simulink model "all_afc_0001_0365"  (R2026a)
settings: Solver=ode15s  StopTime=simTime  FixedStep=5e-05  RelTol=1e-06  AbsTol=1e-06
undefined symbols (not defined in the file): AF_sensor_tol, fault_time, fuel_inj_tol, MAF_sensor_tol, measureTime, simTime, spec_num
(part 1 of 3)
Description:
  | Modeling Engine Timing Using Triggered Subsystems
  | 
  | This example presents a model of a four-cylinder spark ignition engine
  | and demonstrates Simulink(R) capabilities to model an internal combustion
  | engine from the throttle to the crankshaft output. We used well-defined
  | physical principles supplemented, where appropriate, with empirical
  | relationships that describe the systems dynamic behavior without
  | introducing unnecessary complexity.
settings Model: ExtModeTrigMode=oneshot  ExtModeArmWhenConnect=off  ExtModeAutoUpdateStatusClock=off  Creator=The MathWorks Inc.  LastModifiedBy=harry_31916
settings SolverCC: ConsecutiveZCsStepRelTol=2.8421709430404e-13
settings DataIOCC: ExternalInput=[t__,u__]  InitialState=[]  LoadExternalInput=on  SaveFormat=StructureWithTime  SignalLoggingSaveFormat=ModelDataLogs  StateSaveName=x  SignalLoggingName=sldemo_engine_output
settings OptimizationCC: BooleanDataType=off  InitFltsAndDblsToZero=on  BufferReusableBoundary=off
settings DebuggingCC: SignalInfNanChecking=warning  SaveWithParameterizedLinksMsg=none  UnderspecifiedInitializationDetection=Classic  SignalResolutionControl=TryResolveAllWithWarning  InheritedTsInSrcMsg=none  MultiTaskDSMMsg=warning  MultiTaskCondExecSysMsg=none  SigSpecEnsureSampleTimeMsg=none  IntegerOverflowMsg=none  ParameterPrecisionLossMsg=none  UniqueDataStoreMsg=warning  IntegerSaturationMsg=none
settings HardwareCC: ProdHWDeviceType=32-bit Generic
settings GRTTargetCC: TargetFcnLib=ansi_tfl_tmw.mat  CombineOutputUpdateFcns=off  GRTInterface=on
settings ConfigComp: CovMetricSettings=d

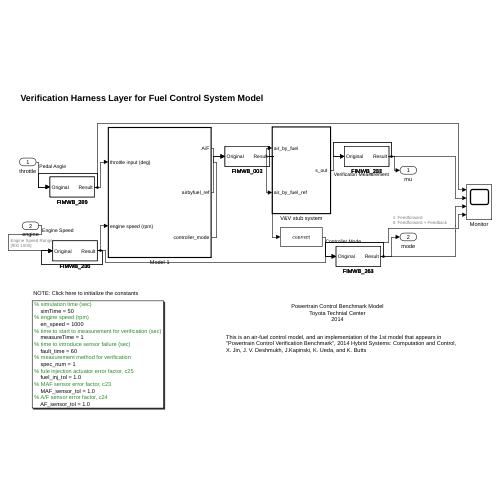
[thumbnail: Simulink's stored preview of the top-level diagram]
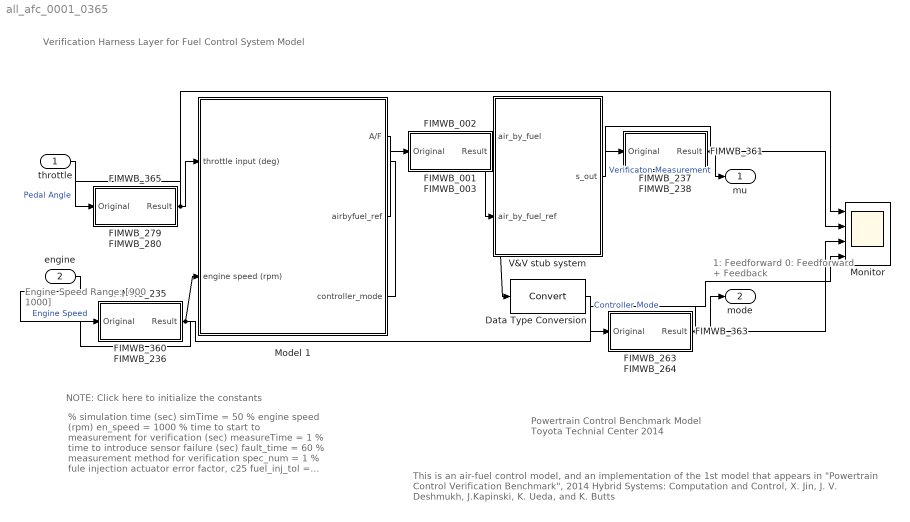
== system all_afc_0001_0365 ==
  note: 1: Feedforward
      | 0: Feedforward + Feedback
  note: NOTE: Click here to initialize the constants
  note: This is an air-fuel control model, and an implementation of the 1st model that appears in
      | "Powertrain Control Verification Benchmark", 2014 Hybrid Systems: Computation and Control,
      | X. Jin, J. V. Deshmukh, J.Kapinski, K. Ueda, and K. Butts
  note: % simulation time (sec)
      |     simTime = 50
      | % engine speed (rpm)
      |     en_speed = 1000
      | % time to start to measurement for verification (sec)
      |     measureTime = 1
      | % time to introduce sensor failure (sec)
      |     fault_time = 60
      | % measurement method for verification
      |     spec_num = 1
      | % fule injection actuator error factor, c25
      |     fuel_inj_tol = 1.0
      | % MAF sensor error factor, c23
      |     MAF_sensor_tol = 1.0
      | % A/F sensor error factor, c24
      |     AF_sensor_tol = 1.0
  note: Engine Speed Range:
      | [900 1000]
  note: Powertrain Control Benchmark Model
      | Toyota Technial Center
      | 2014
  note: Verification Harness Layer for Fuel Control System Model
  throttle : Inport  Interpolate=off
  engine : Inport  Port=2  Interpolate=off
  Data Type Conversion : DataTypeConversion  SaturateOnIntegerOverflow=off  RndMeth=Floor
  FIMWB_001 : Subsystem  Tag=fimwb.fault.1
  FIMWB_002 : Subsystem  Tag=fimwb.fault.2
  FIMWB_003 : Subsystem  Tag=fimwb.fault.3
  FIMWB_235 : Subsystem  Tag=fimwb.fault.235
  FIMWB_236 : Subsystem  Tag=fimwb.fault.236
  FIMWB_237 : Subsystem  Tag=fimwb.fault.237
  FIMWB_238 : Subsystem  Tag=fimwb.fault.238
  FIMWB_263 : Subsystem  Tag=fimwb.fault.263
  FIMWB_264 : Subsystem  Tag=fimwb.fault.264
  FIMWB_279 : Subsystem  Tag=fimwb.fault.279
  FIMWB_280 : Subsystem  Tag=fimwb.fault.280
  FIMWB_360 : Subsystem  Tag=fimwb.fault.360
  FIMWB_361 : Subsystem  Tag=fimwb.fault.361
  FIMWB_363 : Subsystem  Tag=fimwb.fault.363
  FIMWB_365 : Subsystem  Tag=fimwb.fault.365
  Model 1 : Subsystem  Priority=1  TreatAsAtomicUnit=on
  "Monitor " : Scope  NumInputPorts=4
      settings: TimeSpan=50  ActiveDisplayYMinimum=0  ActiveDisplayYMaximum=55
  V&V stub system : Subsystem  TreatAsAtomicUnit=on
  mu : Outport  VectorParamsAs1DForOutWhenUnconnected=off
  mode : Outport  Port=2  VectorParamsAs1DForOutWhenUnconnected=off
  wires:
  engine/1 -> FIMWB_360/1(Original)  "Engine Speed"
  FIMWB_360/1(Result) -> FIMWB_235/1(Original), FIMWB_236/1(Original)
  V&V stub system/1("s_out ") -> FIMWB_361/1(Original)  "Verificaton Measurement"
  FIMWB_361/1(Result) -> FIMWB_237/1(Original), FIMWB_238/1(Original)
  Data Type Conversion/1 -> FIMWB_363/1(Original)  "Controller Mode"
  FIMWB_363/1(Result) -> FIMWB_263/1(Original), FIMWB_264/1(Original)
  throttle/1 -> FIMWB_365/1(Original)  "Pedal Angle"
  FIMWB_365/1(Result) -> FIMWB_279/1(Original), FIMWB_280/1(Original)
  Model 1/1(A/F) -> FIMWB_001/1(Original)
  FIMWB_001/1(Result) -> V&V stub system/1("air_by_fuel ")
  Model 1/2(airbyfuel_ref) -> FIMWB_002/1(Original)
  FIMWB_002/1(Result) -> V&V stub system/2(air_by_fuel_ref)
  Model 1/3(controller_mode) -> FIMWB_003/1(Original)
  FIMWB_003/1(Result) -> Data Type Conversion/1
  FIMWB_235/1(Result) -> "Monitor "/4
  FIMWB_236/1(Result) -> Model 1/2(engine speed (rpm))
  FIMWB_237/1(Result) -> mu/1
  FIMWB_238/1(Result) -> "Monitor "/2
  FIMWB_263/1(Result) -> "Monitor "/3
  FIMWB_264/1(Result) -> mode/1
  FIMWB_279/1(Result) -> "Monitor "/1
  FIMWB_280/1(Result) -> Model 1/1(throttle input (deg))

== system all_afc_0001_0365/FIMWB_001 ==
  Original : Inport
  Result : Outport
  wires:
  Original/1 -> Result/1

== system all_afc_0001_0365/FIMWB_002 ==
  Original : Inport
  Result : Outport
  wires:
  Original/1 -> Result/1

== system all_afc_0001_0365/FIMWB_003 ==
  Original : Inport
  Result : Outport
  wires:
  Original/1 -> Result/1

== system all_afc_0001_0365/FIMWB_235 ==
  Original : Inport
  Result : Outport
  wires:
  Original/1 -> Result/1

== system all_afc_0001_0365/FIMWB_236 ==
  Original : Inport
  Result : Outport
  wires:
  Original/1 -> Result/1

== system all_afc_0001_0365/FIMWB_237 ==
  Original : Inport
  Result : Outport
  wires:
  Original/1 -> Result/1

== system all_afc_0001_0365/FIMWB_238 ==
  Original : Inport
  Result : Outport
  wires:
  Original/1 -> Result/1

== system all_afc_0001_0365/FIMWB_263 ==
  Original : Inport
  Result : Outport
  wires:
  Original/1 -> Result/1

== system all_afc_0001_0365/FIMWB_264 ==
  Original : Inport
  Result : Outport
  wires:
  Original/1 -> Result/1

== system all_afc_0001_0365/FIMWB_279 ==
  Original : Inport
  Result : Outport
  wires:
  Original/1 -> Result/1

== system all_afc_0001_0365/FIMWB_280 ==
  Original : Inport
  Result : Outport
  wires:
  Original/1 -> Result/1

== system all_afc_0001_0365/FIMWB_360 ==
  Original : Inport
  Result : Outport
  wires:
  Original/1 -> Result/1

== system all_afc_0001_0365/FIMWB_361 ==
  Original : Inport
  Result : Outport
  wires:
  Original/1 -> Result/1

== system all_afc_0001_0365/FIMWB_363 ==
  Original : Inport
  Result : Outport
  wires:
  Original/1 -> Result/1

== system all_afc_0001_0365/FIMWB_365 ==
  Original : Inport
  Result : Outport
  wires:
  Original/1 -> Result/1

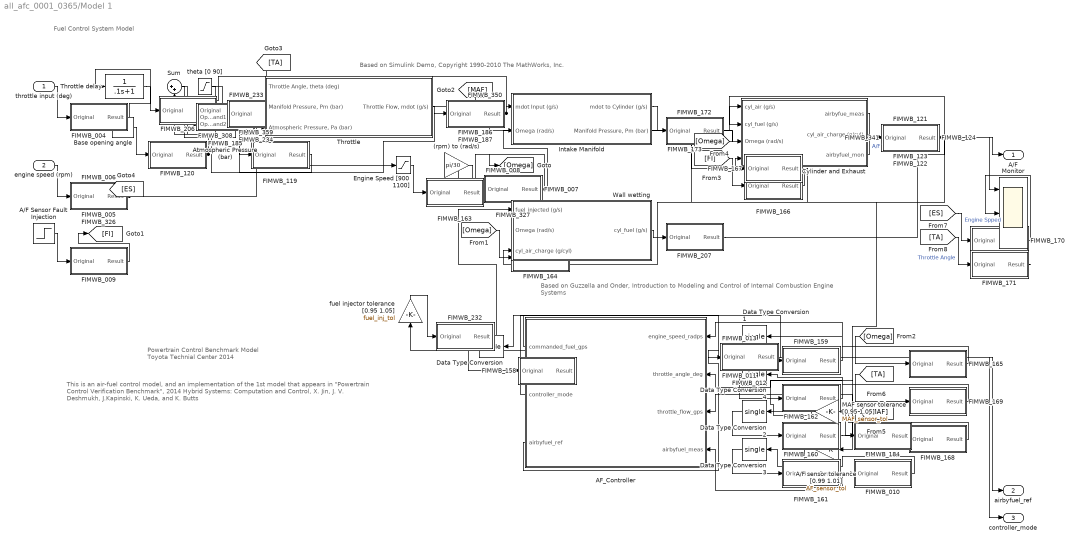
== system all_afc_0001_0365/Model 1 ==
  note: Based on Simulink Demo, Copyright 1990-2010 The MathWorks, Inc.
  note: Based on Guzzella and Onder, Introduction to Modeling and Control of Internal Combustion Engine Systems
  note: Fuel Control System Model
  note: This is an air-fuel control model, and an implementation of the 1st model that appears in
      | "Powertrain Control Verification Benchmark", 2014 Hybrid Systems: Computation and Control,
      | X. Jin, J. V. Deshmukh, J.Kapinski, K. Ueda, and K. Butts
  note: Powertrain Control Benchmark Model
      | Toyota Technial Center
      | 2014
  throttle input (deg) : Inport  Description=[0, 81.2]
      settings: AttributesFormatString=%<Description>
  engine speed (rpm) : Inport  Description=[900,1100]  Port=2
      settings: AttributesFormatString=%<Description>
  (rpm) to (rad/s) : Gain  Gain=pi/30
  A/F Sensor Fault Injection : Step  Time=fault_time  SampleTime=0
      settings: AttributesFormatString=1: Failure\n0: Normal
  A/F sensor tolerance [0.99 1.01] : Gain  Gain=AF_sensor_tol
  AF_Controller : Subsystem  TreatAsAtomicUnit=on
  Atmospheric Pressure (bar) : Constant
  Base opening angle : Constant  Value=8.8
  Cylinder and Exhaust : Subsystem
  Data Type Conversion : DataTypeConversion  OutDataTypeStr=double  SaturateOnIntegerOverflow=off  RndMeth=Floor
  Data Type Conversion{1..4} (4 alike) : DataTypeConversion  OutDataTypeStr=single  SaturateOnIntegerOverflow=off  RndMeth=Floor
  Engine Speed [900 1100] : Saturate  UpperLimit=1100  LowerLimit=900
  FIMWB_004 : Subsystem  Tag=fimwb.fault.4
  FIMWB_005 : Subsystem  Tag=fimwb.fault.5
  FIMWB_006 : Subsystem  Tag=fimwb.fault.6
  FIMWB_007 : Subsystem  Tag=fimwb.fault.7
  FIMWB_008 : Subsystem  Tag=fimwb.fault.8
  FIMWB_009 : Subsystem  Tag=fimwb.fault.9
  FIMWB_010 : Subsystem  Tag=fimwb.fault.10
  FIMWB_011 : Subsystem  Tag=fimwb.fault.11
  FIMWB_012 : Subsystem  Tag=fimwb.fault.12
  FIMWB_013 : Subsystem  Tag=fimwb.fault.13
  FIMWB_119 : Subsystem  Tag=fimwb.fault.119
  FIMWB_120 : Subsystem  Tag=fimwb.fault.120
  FIMWB_121 : Subsystem  Tag=fimwb.fault.121
  FIMWB_122 : Subsystem  Tag=fimwb.fault.122
  FIMWB_123 : Subsystem  Tag=fimwb.fault.123
  FIMWB_124 : Subsystem  Tag=fimwb.fault.124
  FIMWB_158 : Subsystem  Tag=fimwb.fault.158
  FIMWB_159 : Subsystem  Tag=fimwb.fault.159
  FIMWB_160 : Subsystem  Tag=fimwb.fault.160
  FIMWB_161 : Subsystem  Tag=fimwb.fault.161
  FIMWB_162 : Subsystem  Tag=fimwb.fault.162
  FIMWB_163 : Subsystem  Tag=fimwb.fault.163
  FIMWB_164 : Subsystem  Tag=fimwb.fault.164
  FIMWB_165 : Subsystem  Tag=fimwb.fault.165
  FIMWB_166 : Subsystem  Tag=fimwb.fault.166
  FIMWB_167 : Subsystem  Tag=fimwb.fault.167
  FIMWB_168 : Subsystem  Tag=fimwb.fault.168
  FIMWB_169 : Subsystem  Tag=fimwb.fault.169
  FIMWB_170 : Subsystem  Tag=fimwb.fault.170
  FIMWB_171 : Subsystem  Tag=fimwb.fault.171
  FIMWB_172 : Subsystem  Tag=fimwb.fault.172
  FIMWB_173 : Subsystem  Tag=fimwb.fault.173
  FIMWB_184 : Subsystem  Tag=fimwb.fault.184
  FIMWB_185 : Subsystem  Tag=fimwb.fault.185
  FIMWB_186 : Subsystem  Tag=fimwb.fault.186
  FIMWB_187 : Subsystem  Tag=fimwb.fault.187
  FIMWB_206 : Subsystem  Tag=fimwb.fault.206
  FIMWB_207 : Subsystem  Tag=fimwb.fault.207
  FIMWB_232 : Subsystem  Tag=fimwb.fault.232
  FIMWB_233 : Subsystem  Tag=fimwb.fault.233
  FIMWB_234 : Subsystem  Tag=fimwb.fault.234
  FIMWB_308 : Subsystem  Tag=fimwb.fault.308
  FIMWB_326 : Subsystem  Tag=fimwb.fault.326
  FIMWB_327 : Subsystem  Tag=fimwb.fault.327
  FIMWB_341 : Subsystem  Tag=fimwb.fault.341
  FIMWB_350 : Subsystem  Tag=fimwb.fault.350
  FIMWB_359 : Subsystem  Tag=fimwb.fault.359
  Intake Manifold : Subsystem
  MAF sensor tolerance [0.95 1.05] : Gain  Gain=MAF_sensor_tol
  Monitor : Scope  NumInputPorts=3
      settings: TimeSpan=85  ActiveDisplayYMinimum=11.75  ActiveDisplayYMaximum=14.75
  Sum : Sum  Inputs=|++
  Throttle : Subsystem
  Throttle delay : TransferFcn  Denominator=[.1 1]
  Wall wetting : Subsystem
  fuel injector tolerance [0.95 1.05] : Gain  Gain=fuel_inj_tol
  theta [0 90] : Saturate  UpperLimit=90  LowerLimit=0
  A/F : Outport  VectorParamsAs1DForOutWhenUnconnected=off
  airbyfuel_ref : Outport  Port=2  VectorParamsAs1DForOutWhenUnconnected=off
  controller_mode : Outport  Port=3  VectorParamsAs1DForOutWhenUnconnected=off
  wires:
  Sum/1 -> FIMWB_308/1(Original)
  engine speed (rpm)/1 -> FIMWB_326/1(Original)
  FIMWB_326/1(Result) -> FIMWB_005/1(Original), FIMWB_006/1(Original)
  (rpm) to (rad/s)/1 -> FIMWB_327/1(Original)
  FIMWB_327/1(Result) -> FIMWB_007/1(Original), FIMWB_008/1(Original)
  Cylinder and Exhaust/3("airbyfuel_mon ") -> FIMWB_341/1(Original)  "A/F"
  FIMWB_341/1(Result) -> FIMWB_123/1(Original), FIMWB_124/1(Original)
  Throttle/1("Throttle Flow, mdot (g/s)") -> FIMWB_350/1(Original)
  FIMWB_350/1(Result) -> FIMWB_186/1(Original), FIMWB_187/1(Original)
  theta [0 90]/1 -> FIMWB_359/1(Original)
  FIMWB_359/1(Result) -> FIMWB_233/1(Original), FIMWB_234/1(Original)
  throttle input (deg)/1 -> FIMWB_004/1(Original)
  FIMWB_004/1(Result) -> Throttle delay/1
  FIMWB_005/1(Result) -> Engine Speed [900 1100]/1
  FIMWB_006/1(Result) -> [ES]
  FIMWB_007/1(Result) -> [Omega]
  FIMWB_008/1(Result) -> Intake Manifold/2(Omega (rad/s))
  A/F Sensor Fault Injection/1 -> FIMWB_009/1(Original)
  FIMWB_009/1(Result) -> [FI]
  A/F sensor tolerance [0.99 1.01]/1 -> FIMWB_010/1(Original)
  FIMWB_010/1(Result) -> Data Type Conversion3/1
  AF_Controller/1(commanded_fuel_gps) -> FIMWB_011/1(Original)
  FIMWB_011/1(Result) -> Data Type Conversion/1
  AF_Controller/2(controller_mode) -> FIMWB_012/1(Original)
  FIMWB_012/1(Result) -> controller_mode/1
  AF_Controller/3(airbyfuel_ref) -> FIMWB_013/1(Original)
  FIMWB_013/1(Result) -> airbyfuel_ref/1
  Atmospheric Pressure (bar)/1 -> FIMWB_119/1(Original)
  FIMWB_119/1(Result) -> Throttle/3("Atmospheric Pressure, Pa (bar) ")
  Base opening angle/1 -> FIMWB_120/1(Original)
  FIMWB_120/1(Result) -> Sum/2, FIMWB_308/3(Operand2)
  Cylinder and Exhaust/1(airbyfue_meas) -> FIMWB_121/1(Original)
  FIMWB_121/1(Result) -> A/F sensor tolerance [0.99 1.01]/1
  Cylinder and Exhaust/2(cyl_air_charge (g/cyl)) -> FIMWB_122/1(Original)
  FIMWB_122/1(Result) -> Wall wetting/3(cyl_air_charge (g/cyl))
  FIMWB_123/1(Result) -> Monitor/1
  FIMWB_124/1(Result) -> A/F/1
  Data Type Conversion/1 -> FIMWB_158/1(Original)
  FIMWB_158/1(Result) -> fuel injector tolerance [0.95 1.05]/1
  Data Type Conversion1/1 -> FIMWB_159/1(Original)
  FIMWB_159/1(Result) -> AF_Controller/1(engine_speed_radps)
  Data Type Conversion2/1 -> FIMWB_160/1(Original)
  FIMWB_160/1(Result) -> AF_Controller/3(throttle_flow_gps)
  Data Type Conversion3/1 -> FIMWB_161/1(Original)
  FIMWB_161/1(Result) -> AF_Controller/4(airbyfuel_meas)
  Data Type Conversion4/1 -> FIMWB_162/1(Original)
  FIMWB_162/1(Result) -> AF_Controller/2(throttle_angle_deg)
  Engine Speed [900 1100]/1 -> FIMWB_163/1(Original)
  FIMWB_163/1(Result) -> (rpm) to (rad/s)/1
  [Omega] -> FIMWB_164/1(Original)
  FIMWB_164/1(Result) -> Wall wetting/2(Omega (rad/s))
  [Omega] -> FIMWB_165/1(Original)
  FIMWB_165/1(Result) -> Data Type Conversion1/1
  [FI] -> FIMWB_166/1(Original)
  FIMWB_166/1(Result) -> Cylinder and Exhaust/4(SensorFault)
  [Omega] -> FIMWB_167/1(Original)
  FIMWB_167/1(Result) -> Cylinder and Exhaust/3(Omega (rad/s))
  [MAF] -> FIMWB_168/1(Original)
  FIMWB_168/1(Result) -> MAF sensor tolerance [0.95 1.05]/1
  [TA] -> FIMWB_169/1(Original)
  FIMWB_169/1(Result) -> Data Type Conversion4/1
  [ES] -> FIMWB_170/1(Original)  "Engine Spped"
  FIMWB_170/1(Result) -> Monitor/2
  [TA] -> FIMWB_171/1(Original)  "Throttle Angle"
  FIMWB_171/1(Result) -> Monitor/3
  Intake Manifold/1(mdot to Cylinder (g/s)) -> FIMWB_172/1(Original)
  FIMWB_172/1(Result) -> Cylinder and Exhaust/1(cyl_air (g/s))
  Intake Manifold/2("Manifold Pressure, Pm (bar)") -> FIMWB_173/1(Original)
  FIMWB_173/1(Result) -> Throttle/2("Manifold Pressure, Pm (bar)")
  MAF sensor tolerance [0.95 1.05]/1 -> FIMWB_184/1(Original)
  FIMWB_184/1(Result) -> Data Type Conversion2/1
  FIMWB_308/1(Result) -> FIMWB_185/1(Original)
  FIMWB_185/1(Result) -> theta [0 90]/1
  FIMWB_186/1(Result) -> [MAF]
  FIMWB_187/1(Result) -> Intake Manifold/1(mdot Input (g/s))
  Throttle delay/1 -> FIMWB_206/1(Original)
  FIMWB_206/1(Result) -> Sum/1, FIMWB_308/2(Operand1)
  Wall wetting/1(cyl_fuel (g/s)) -> FIMWB_207/1(Original)
  FIMWB_207/1(Result) -> Cylinder and Exhaust/2(cyl_fuel (g/s))
  fuel injector tolerance [0.95 1.05]/1 -> FIMWB_232/1(Original)
  FIMWB_232/1(Result) -> Wall wetting/1(fuel_injected (g/s))
  FIMWB_233/1(Result) -> [TA]
  FIMWB_234/1(Result) -> Throttle/1("Throttle Angle, theta (deg)")

== system all_afc_0001_0365/V&V stub system ==
  "air_by_fuel " : Inport  OutDataTypeStr=double
  air_by_fuel_ref : Inport  Port=2
  Calcuate Error : Subsystem  Priority=20  TreatAsAtomicUnit=on
  Constant : Constant  Value=0.5
  Data Type Conversion : DataTypeConversion  OutDataTypeStr=double  SaturateOnIntegerOverflow=off  RndMeth=Floor
  FIMWB_239 : Subsystem  Tag=fimwb.fault.239
  FIMWB_240 : Subsystem  Tag=fimwb.fault.240
  FIMWB_260 : Subsystem  Tag=fimwb.fault.260
  FIMWB_261 : Subsystem  Tag=fimwb.fault.261
  FIMWB_265 : Subsystem  Tag=fimwb.fault.265
  FIMWB_275 : Subsystem  Tag=fimwb.fault.275
  FIMWB_276 : Subsystem  Tag=fimwb.fault.276
  MeasureOn : Step  Time=measureTime  SampleTime=0
  Relational Operator : RelationalOperator  Operator=>  OutDataTypeStr=boolean  InputSameDT=off
  spec_num : Constant  Value=spec_num  OutDataTypeStr=uint8
  "s_out " : Outport  VectorParamsAs1DForOutWhenUnconnected=off
  wires:
  Relational Operator/1 -> Calcuate Error/Enable
  "air_by_fuel "/1 -> FIMWB_239/1(Original)
  FIMWB_239/1(Result) -> Calcuate Error/1("air_by_fuel ")
  Calcuate Error/1("s_out ") -> FIMWB_240/1(Original)
  FIMWB_240/1(Result) -> "s_out "/1
  Constant/1 -> FIMWB_260/1(Original)
  FIMWB_260/1(Result) -> Relational Operator/2
  MeasureOn/1 -> FIMWB_261/1(Original)
  FIMWB_261/1(Result) -> Relational Operator/1
  spec_num/1 -> FIMWB_265/1(Original)
  FIMWB_265/1(Result) -> Calcuate Error/2(spec_num)
  air_by_fuel_ref/1 -> FIMWB_275/1(Original)
  FIMWB_275/1(Result) -> Data Type Conversion/1
  Data Type Conversion/1 -> FIMWB_276/1(Original)
  FIMWB_276/1(Result) -> Calcuate Error/3(air_by_fuel_ref)

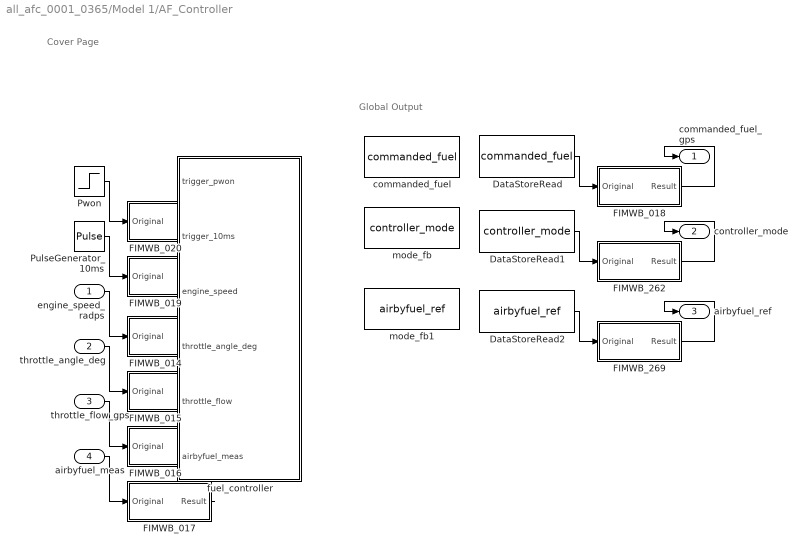
== system all_afc_0001_0365/Model 1/AF_Controller ==
  note: Global Output
  note: Cover Page
  engine_speed_radps : Inport
  throttle_angle_deg : Inport  Port=2
  throttle_flow_gps : Inport  Port=3
  airbyfuel_meas : Inport  Port=4
  DataStoreRead : DataStoreRead  Priority=2  DataStoreName=commanded_fuel  IndexOptions=Index vector (dialog)  Indices=1  OutputSizes=1
  DataStoreRead1 : DataStoreRead  Priority=2  DataStoreName=controller_mode  IndexOptions=Index vector (dialog)  Indices=1  OutputSizes=1
  DataStoreRead2 : DataStoreRead  Priority=2  DataStoreName=airbyfuel_ref  IndexOptions=Index vector (dialog)  Indices=1  OutputSizes=1
  FIMWB_014 : Subsystem  Tag=fimwb.fault.14
  FIMWB_015 : Subsystem  Tag=fimwb.fault.15
  FIMWB_016 : Subsystem  Tag=fimwb.fault.16
  FIMWB_017 : Subsystem  Tag=fimwb.fault.17
  FIMWB_018 : Subsystem  Tag=fimwb.fault.18
  FIMWB_019 : Subsystem  Tag=fimwb.fault.19
  FIMWB_020 : Subsystem  Tag=fimwb.fault.20
  FIMWB_262 : Subsystem  Tag=fimwb.fault.262
  FIMWB_269 : Subsystem  Tag=fimwb.fault.269
  PulseGenerator_10ms : DiscretePulseGenerator  PulseType=Time based  Period=0.01  PulseWidth=50  PhaseDelay=0.01
  Pwon : Step  Time=0.001  SampleTime=0
  commanded_fuel : DataStoreMemory  DataStoreName=commanded_fuel  InitialValue=0.1726  ShowAdditionalParam=off  OutDataTypeStr=single
      settings: AttributesFormatString=commanded_fuel
  fuel_controller : Subsystem  Priority=1  TreatAsAtomicUnit=on
      settings: AttributesFormatString=Priority = %<Priority>
  mode_fb : DataStoreMemory  DataStoreName=controller_mode  ShowAdditionalParam=off  OutDataTypeStr=boolean
      settings: AttributesFormatString=controller_mode
  mode_fb1 : DataStoreMemory  DataStoreName=airbyfuel_ref  ShowAdditionalParam=off  OutDataTypeStr=single
  commanded_fuel_gps : Outport  VectorParamsAs1DForOutWhenUnconnected=off
  controller_mode : Outport  Port=2  VectorParamsAs1DForOutWhenUnconnected=off
  airbyfuel_ref : Outport  Port=3  VectorParamsAs1DForOutWhenUnconnected=off
  wires:
  engine_speed_radps/1 -> FIMWB_014/1(Original)
  FIMWB_014/1(Result) -> fuel_controller/3(engine_speed)
  throttle_angle_deg/1 -> FIMWB_015/1(Original)
  FIMWB_015/1(Result) -> fuel_controller/4(throttle_angle_deg)
  throttle_flow_gps/1 -> FIMWB_016/1(Original)
  FIMWB_016/1(Result) -> fuel_controller/5(throttle_flow)
  airbyfuel_meas/1 -> FIMWB_017/1(Original)
  FIMWB_017/1(Result) -> fuel_controller/6(airbyfuel_meas)
  DataStoreRead/1 -> FIMWB_018/1(Original)
  FIMWB_018/1(Result) -> commanded_fuel_gps/1
  PulseGenerator_10ms/1 -> FIMWB_019/1(Original)
  FIMWB_019/1(Result) -> fuel_controller/2(trigger_10ms)
  Pwon/1 -> FIMWB_020/1(Original)
  FIMWB_020/1(Result) -> fuel_controller/1(trigger_pwon)
  DataStoreRead1/1 -> FIMWB_262/1(Original)
  FIMWB_262/1(Result) -> controller_mode/1
  DataStoreRead2/1 -> FIMWB_269/1(Original)
  FIMWB_269/1(Result) -> airbyfuel_ref/1

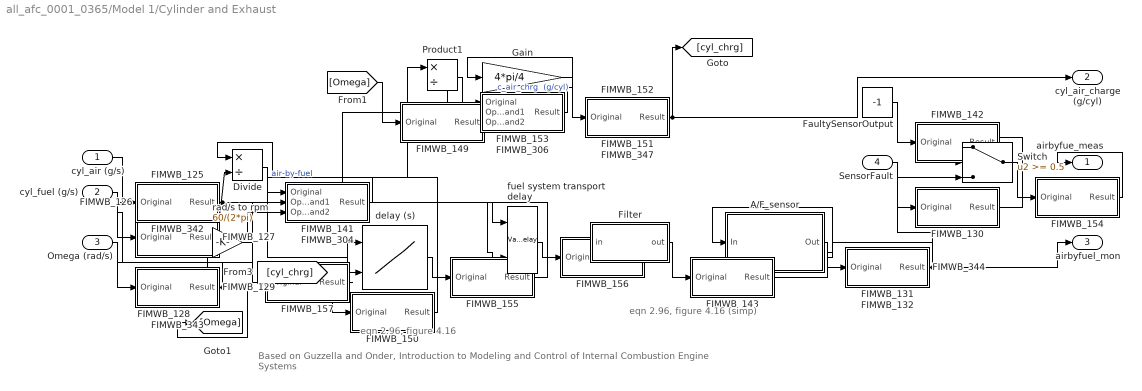
== system all_afc_0001_0365/Model 1/Cylinder and Exhaust ==
  note: Based on Guzzella and Onder, Introduction to Modeling and Control of Internal Combustion Engine Systems
  note: eqn 2.96, figure 4.16
  note: eqn 2.96, figure 4.16 (simp)
  cyl_air (g/s) : Inport
  cyl_fuel (g/s) : Inport  Port=2
  Omega (rad/s) : Inport  Port=3
  SensorFault : Inport  Port=4
  A/F_sensor : Subsystem
  Divide : Product  Inputs=*/
  FIMWB_125 : Subsystem  Tag=fimwb.fault.125
  FIMWB_126 : Subsystem  Tag=fimwb.fault.126
  FIMWB_127 : Subsystem  Tag=fimwb.fault.127
  FIMWB_128 : Subsystem  Tag=fimwb.fault.128
  FIMWB_129 : Subsystem  Tag=fimwb.fault.129
  FIMWB_130 : Subsystem  Tag=fimwb.fault.130
  FIMWB_131 : Subsystem  Tag=fimwb.fault.131
  FIMWB_132 : Subsystem  Tag=fimwb.fault.132
  FIMWB_141 : Subsystem  Tag=fimwb.fault.141
  FIMWB_142 : Subsystem  Tag=fimwb.fault.142
  FIMWB_143 : Subsystem  Tag=fimwb.fault.143
  FIMWB_149 : Subsystem  Tag=fimwb.fault.149
  FIMWB_150 : Subsystem  Tag=fimwb.fault.150
  FIMWB_151 : Subsystem  Tag=fimwb.fault.151
  FIMWB_152 : Subsystem  Tag=fimwb.fault.152
  FIMWB_153 : Subsystem  Tag=fimwb.fault.153
  FIMWB_154 : Subsystem  Tag=fimwb.fault.154
  FIMWB_155 : Subsystem  Tag=fimwb.fault.155
  FIMWB_156 : Subsystem  Tag=fimwb.fault.156
  FIMWB_157 : Subsystem  Tag=fimwb.fault.157
  FIMWB_304 : Subsystem  Tag=fimwb.fault.304
  FIMWB_306 : Subsystem  Tag=fimwb.fault.306
  FIMWB_342 : Subsystem  Tag=fimwb.fault.342
  FIMWB_343 : Subsystem  Tag=fimwb.fault.343
  FIMWB_344 : Subsystem  Tag=fimwb.fault.344
  FIMWB_347 : Subsystem  Tag=fimwb.fault.347
  FaultySensorOutput : Constant  Value=-1
  Filter : Subsystem
  Gain : Gain  Gain=4*pi/4
  Product1 : Product  Inputs=*/  RndMeth=Zero
  Switch : Switch  Threshold=0.5  SaturateOnIntegerOverflow=off  InputSameDT=off
  delay (s) : Lookup_n-D  BreakpointsForDimension1=[800,1000,1500,2000,3000]  BreakpointsForDimension2=[0.05,0.15,0.2,0.25]  Table=reshape([0.8,0.6,0.4,0.3,0.2,0.4,0.3,0.2,0.2,0.2,0.3,0.25,0.2,0.2,0.2,0.25,0.2,0.2,0.2,0.2],5,4)  UseLastTableValue=on  RndMeth=Simplest
      settings: InputPortMap=u0,u1
  fuel system transport delay : VariableTransportDelay  VariableDelayType=Variable transport delay  MaximumDelay=10  InitialOutput=14.7  MaximumPoints=20480
  rad/s to rpm : Gain  Gain=60/(2*pi)
  airbyfue_meas : Outport  VectorParamsAs1DForOutWhenUnconnected=off
  cyl_air_charge (g/cyl) : Outport  Port=2  VectorParamsAs1DForOutWhenUnconnected=off
  "airbyfuel_mon " : Outport  Port=3  VectorParamsAs1DForOutWhenUnconnected=off
  wires:
  Divide/1 -> FIMWB_304/1(Original)  "air-by-fuel"
  Product1/1 -> FIMWB_306/1(Original)
  cyl_air (g/s)/1 -> FIMWB_342/1(Original)
  FIMWB_342/1(Result) -> FIMWB_125/1(Original), FIMWB_126/1(Original)
  Omega (rad/s)/1 -> FIMWB_343/1(Original)
  FIMWB_343/1(Result) -> FIMWB_128/1(Original), FIMWB_129/1(Original)
  A/F_sensor/1(Out) -> FIMWB_344/1(Original)
  FIMWB_344/1(Result) -> FIMWB_131/1(Original), FIMWB_132/1(Original)
  Gain/1 -> FIMWB_347/1(Original)  "c_air_chrg  (g/cyl)"
  FIMWB_347/1(Result) -> FIMWB_151/1(Original), FIMWB_152/1(Original)
  FIMWB_125/1(Result) -> Divide/1, FIMWB_304/2(Operand1)
  FIMWB_126/1(Result) -> Product1/1, FIMWB_306/2(Operand1)
  cyl_fuel (g/s)/1 -> FIMWB_127/1(Original)
  FIMWB_127/1(Result) -> Divide/2, FIMWB_304/3(Operand2)
  FIMWB_128/1(Result) -> [Omega]
  FIMWB_129/1(Result) -> rad/s to rpm/1
  SensorFault/1 -> FIMWB_130/1(Original)
  FIMWB_130/1(Result) -> Switch/2
  FIMWB_131/1(Result) -> Switch/3
  FIMWB_132/1(Result) -> "airbyfuel_mon "/1
  FIMWB_304/1(Result) -> FIMWB_141/1(Original)
  FIMWB_141/1(Result) -> fuel system transport delay/1
  FaultySensorOutput/1 -> FIMWB_142/1(Original)
  FIMWB_142/1(Result) -> Switch/1
  Filter/1(out) -> FIMWB_143/1(Original)
  FIMWB_143/1(Result) -> A/F_sensor/1(In)
  [Omega] -> FIMWB_149/1(Original)
  FIMWB_149/1(Result) -> Product1/2, FIMWB_306/3(Operand2)
  [cyl_chrg] -> FIMWB_150/1(Original)
  FIMWB_150/1(Result) -> delay (s)/2
  FIMWB_151/1(Result) -> [cyl_chrg]
  FIMWB_152/1(Result) -> cyl_air_charge (g/cyl)/1
  FIMWB_306/1(Result) -> FIMWB_153/1(Original)
  FIMWB_153/1(Result) -> Gain/1
  Switch/1 -> FIMWB_154/1(Original)
  FIMWB_154/1(Result) -> airbyfue_meas/1
  delay (s)/1 -> FIMWB_155/1(Original)
  FIMWB_155/1(Result) -> fuel system transport delay/2
  fuel system transport delay/1 -> FIMWB_156/1(Original)
  FIMWB_156/1(Result) -> Filter/1(in)
  rad/s to rpm/1 -> FIMWB_157/1(Original)
  FIMWB_157/1(Result) -> delay (s)/1

== system all_afc_0001_0365/Model 1/FIMWB_004 ==
  Original : Inport
  Result : Outport
  wires:
  Original/1 -> Result/1

== system all_afc_0001_0365/Model 1/FIMWB_005 ==
  Original : Inport
  Result : Outport
  wires:
  Original/1 -> Result/1

== system all_afc_0001_0365/Model 1/FIMWB_006 ==
  Original : Inport
  Result : Outport
  wires:
  Original/1 -> Result/1

== system all_afc_0001_0365/Model 1/FIMWB_007 ==
  Original : Inport
  Result : Outport
  wires:
  Original/1 -> Result/1

== system all_afc_0001_0365/Model 1/FIMWB_008 ==
  Original : Inport
  Result : Outport
  wires:
  Original/1 -> Result/1

== system all_afc_0001_0365/Model 1/FIMWB_009 ==
  Original : Inport
  Result : Outport
  wires:
  Original/1 -> Result/1

== system all_afc_0001_0365/Model 1/FIMWB_010 ==
  Original : Inport
  Result : Outport
  wires:
  Original/1 -> Result/1

== system all_afc_0001_0365/Model 1/FIMWB_011 ==
  Original : Inport
  Result : Outport
  wires:
  Original/1 -> Result/1

== system all_afc_0001_0365/Model 1/FIMWB_012 ==
  Original : Inport
  Result : Outport
  wires:
  Original/1 -> Result/1

== system all_afc_0001_0365/Model 1/FIMWB_013 ==
  Original : Inport
  Result : Outport
  wires:
  Original/1 -> Result/1

== system all_afc_0001_0365/Model 1/FIMWB_119 ==
  Original : Inport
  Result : Outport
  wires:
  Original/1 -> Result/1

== system all_afc_0001_0365/Model 1/FIMWB_120 ==
  Original : Inport
  Result : Outport
  wires:
  Original/1 -> Result/1

== system all_afc_0001_0365/Model 1/FIMWB_121 ==
  Original : Inport
  Result : Outport
  wires:
  Original/1 -> Result/1

== system all_afc_0001_0365/Model 1/FIMWB_122 ==
  Original : Inport
  Result : Outport
  wires:
  Original/1 -> Result/1

== system all_afc_0001_0365/Model 1/FIMWB_123 ==
  Original : Inport
  Result : Outport
  wires:
  Original/1 -> Result/1

== system all_afc_0001_0365/Model 1/FIMWB_124 ==
  Original : Inport
  Result : Outport
  wires:
  Original/1 -> Result/1

== system all_afc_0001_0365/Model 1/FIMWB_158 ==
  Original : Inport
  Result : Outport
  wires:
  Original/1 -> Result/1

== system all_afc_0001_0365/Model 1/FIMWB_159 ==
  Original : Inport
  Result : Outport
  wires:
  Original/1 -> Result/1

== system all_afc_0001_0365/Model 1/FIMWB_160 ==
  Original : Inport
  Result : Outport
  wires:
  Original/1 -> Result/1

== system all_afc_0001_0365/Model 1/FIMWB_161 ==
  Original : Inport
  Result : Outport
  wires:
  Original/1 -> Result/1

== system all_afc_0001_0365/Model 1/FIMWB_162 ==
  Original : Inport
  Result : Outport
  wires:
  Original/1 -> Result/1

== system all_afc_0001_0365/Model 1/FIMWB_163 ==
  Original : Inport
  Result : Outport
  wires:
  Original/1 -> Result/1

== system all_afc_0001_0365/Model 1/FIMWB_164 ==
  Original : Inport
  Result : Outport
  wires:
  Original/1 -> Result/1

== system all_afc_0001_0365/Model 1/FIMWB_165 ==
  Original : Inport
  Result : Outport
  wires:
  Original/1 -> Result/1

== system all_afc_0001_0365/Model 1/FIMWB_166 ==
  Original : Inport
  Result : Outport
  wires:
  Original/1 -> Result/1

== system all_afc_0001_0365/Model 1/FIMWB_167 ==
  Original : Inport
  Result : Outport
  wires:
  Original/1 -> Result/1

== system all_afc_0001_0365/Model 1/FIMWB_168 ==
  Original : Inport
  Result : Outport
  wires:
  Original/1 -> Result/1

== system all_afc_0001_0365/Model 1/FIMWB_169 ==
  Original : Inport
  Result : Outport
  wires:
  Original/1 -> Result/1

== system all_afc_0001_0365/Model 1/FIMWB_170 ==
  Original : Inport
  Result : Outport
  wires:
  Original/1 -> Result/1

== system all_afc_0001_0365/Model 1/FIMWB_171 ==
  Original : Inport
  Result : Outport
  wires:
  Original/1 -> Result/1

== system all_afc_0001_0365/Model 1/FIMWB_172 ==
  Original : Inport
  Result : Outport
  wires:
  Original/1 -> Result/1

== system all_afc_0001_0365/Model 1/FIMWB_173 ==
  Original : Inport
  Result : Outport
  wires:
  Original/1 -> Result/1

== system all_afc_0001_0365/Model 1/FIMWB_184 ==
  Original : Inport
  Result : Outport
  wires:
  Original/1 -> Result/1

== system all_afc_0001_0365/Model 1/FIMWB_185 ==
  Original : Inport
  Result : Outport
  wires:
  Original/1 -> Result/1

== system all_afc_0001_0365/Model 1/FIMWB_186 ==
  Original : Inport
  Result : Outport
  wires:
  Original/1 -> Result/1

== system all_afc_0001_0365/Model 1/FIMWB_187 ==
  Original : Inport
  Result : Outport
  wires:
  Original/1 -> Result/1

== system all_afc_0001_0365/Model 1/FIMWB_206 ==
  Original : Inport
  Result : Outport
  wires:
  Original/1 -> Result/1

== system all_afc_0001_0365/Model 1/FIMWB_207 ==
  Original : Inport
  Result : Outport
  wires:
  Original/1 -> Result/1

== system all_afc_0001_0365/Model 1/FIMWB_232 ==
  Original : Inport
  Result : Outport
  wires:
  Original/1 -> Result/1

== system all_afc_0001_0365/Model 1/FIMWB_233 ==
  Original : Inport
  Result : Outport
  wires:
  Original/1 -> Result/1

== system all_afc_0001_0365/Model 1/FIMWB_234 ==
  Original : Inport
  Result : Outport
  wires:
  Original/1 -> Result/1

== system all_afc_0001_0365/Model 1/FIMWB_308 ==
  Original : Inport
  Operand1 : Inport  Port=2
  Operand2 : Inport  Port=3
  Unused2 : Terminator
  Unused3 : Terminator
  Result : Outport
  wires:
  Original/1 -> Result/1
  Operand1/1 -> Unused2/1
  Operand2/1 -> Unused3/1

== system all_afc_0001_0365/Model 1/FIMWB_326 ==
  Original : Inport
  Result : Outport
  wires:
  Original/1 -> Result/1

== system all_afc_0001_0365/Model 1/FIMWB_327 ==
  Original : Inport
  Result : Outport
  wires:
  Original/1 -> Result/1

== system all_afc_0001_0365/Model 1/FIMWB_341 ==
  Original : Inport
  Result : Outport
  wires:
  Original/1 -> Result/1

== system all_afc_0001_0365/Model 1/FIMWB_350 ==
  Original : Inport
  Result : Outport
  wires:
  Original/1 -> Result/1

== system all_afc_0001_0365/Model 1/FIMWB_359 ==
  Original : Inport
  Result : Outport
  wires:
  Original/1 -> Result/1

== system all_afc_0001_0365/Model 1/Intake Manifold ==
  note: Intake Manifold Vacuum
  note: Based on Simulink Demo, Copyright 1990-2010 The MathWorks, Inc.
  mdot Input (g/s) : Inport
  Omega (rad/s) : Inport  Port=2
  FIMWB_174 : Subsystem  Tag=fimwb.fault.174
  FIMWB_175 : Subsystem  Tag=fimwb.fault.175
  FIMWB_176 : Subsystem  Tag=fimwb.fault.176
  FIMWB_177 : Subsystem  Tag=fimwb.fault.177
  FIMWB_178 : Subsystem  Tag=fimwb.fault.178
  FIMWB_179 : Subsystem  Tag=fimwb.fault.179
  FIMWB_180 : Subsystem  Tag=fimwb.fault.180
  FIMWB_181 : Subsystem  Tag=fimwb.fault.181
  FIMWB_182 : Subsystem  Tag=fimwb.fault.182
  FIMWB_183 : Subsystem  Tag=fimwb.fault.183
  FIMWB_307 : Subsystem  Tag=fimwb.fault.307
  FIMWB_348 : Subsystem  Tag=fimwb.fault.348
  FIMWB_349 : Subsystem  Tag=fimwb.fault.349
  Gain2 : Gain  Gain=0.9  ParamDataTypeStr=single  OutDataTypeStr=Inherit: Inherit via back propagation  RndMeth=Simplest  SaturateOnIntegerOverflow=on
      settings: AttributesFormatString=pumping tolerance [0.9 1.1]
  Mux : Mux  Inputs=2
  Pumping : Fcn  Expr=-0.366 + 0.08979*u[1]*u[2] - 0.0337*u[2]*u[1]*u[1] + 0.0001*u[1]*u[2]*u[2]
  RT/Vm : Gain  Gain=0.41328  SaturateOnIntegerOverflow=on  OutDataTypeStr=Inherit: Same as input  ParamDataTypeStr=Inherit: Same as input
  Sum : Sum  Inputs=|+-  InputSameDT=on  SaturateOnIntegerOverflow=on  OutDataTypeStr=Inherit: Same as first input
  p0 = 0.543 (bar) : Integrator  InitialCondition=0.982
  mdot to Cylinder (g/s) : Outport  InitialOutput=0  VectorParamsAs1DForOutWhenUnconnected=off
  "Manifold Pressure, Pm (bar)" : Outport  Port=2  InitialOutput=0  VectorParamsAs1DForOutWhenUnconnected=off
  wires:
  Sum/1 -> FIMWB_307/1(Original)
  Gain2/1 -> FIMWB_348/1(Original)
  FIMWB_348/1(Result) -> FIMWB_176/1(Original), FIMWB_177/1(Original)
  p0 = 0.543 (bar)/1 -> FIMWB_349/1(Original)
  FIMWB_349/1(Result) -> FIMWB_182/1(Original), FIMWB_183/1(Original)
  mdot Input (g/s)/1 -> FIMWB_174/1(Original)
  FIMWB_174/1(Result) -> Sum/1, FIMWB_307/2(Operand1)
  Omega (rad/s)/1 -> FIMWB_175/1(Original)
  FIMWB_175/1(Result) -> Mux/2
  FIMWB_176/1(Result) -> Sum/2, FIMWB_307/3(Operand2)
  FIMWB_177/1(Result) -> mdot to Cylinder (g/s)/1
  Mux/1 -> FIMWB_178/1(Original)
  FIMWB_178/1(Result) -> Pumping/1
  Pumping/1 -> FIMWB_179/1(Original)
  FIMWB_179/1(Result) -> Gain2/1
  RT/Vm/1 -> FIMWB_180/1(Original)
  FIMWB_180/1(Result) -> p0 = 0.543 (bar)/1
  FIMWB_307/1(Result) -> FIMWB_181/1(Original)
  FIMWB_181/1(Result) -> RT/Vm/1
  FIMWB_182/1(Result) -> Mux/1
  FIMWB_183/1(Result) -> "Manifold Pressure, Pm (bar)"/1

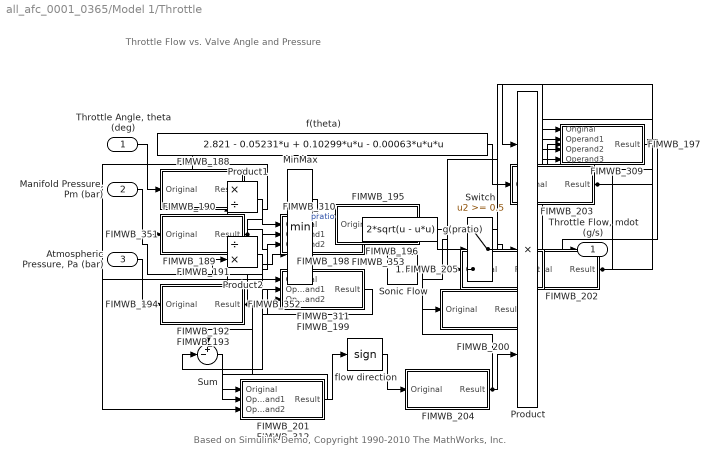
== system all_afc_0001_0365/Model 1/Throttle ==
  note: Throttle Flow vs. Valve Angle and Pressure
  note: Based on Simulink Demo, Copyright 1990-2010 The MathWorks, Inc.
  "Throttle Angle, theta (deg)" : Inport
  "Manifold Pressure, Pm (bar)" : Inport  Port=2
  "Atmospheric Pressure, Pa (bar) " : Inport  Port=3
  FIMWB_188 : Subsystem  Tag=fimwb.fault.188
  FIMWB_189 : Subsystem  Tag=fimwb.fault.189
  FIMWB_190 : Subsystem  Tag=fimwb.fault.190
  FIMWB_191 : Subsystem  Tag=fimwb.fault.191
  FIMWB_192 : Subsystem  Tag=fimwb.fault.192
  FIMWB_193 : Subsystem  Tag=fimwb.fault.193
  FIMWB_194 : Subsystem  Tag=fimwb.fault.194
  FIMWB_195 : Subsystem  Tag=fimwb.fault.195
  FIMWB_196 : Subsystem  Tag=fimwb.fault.196
  FIMWB_197 : Subsystem  Tag=fimwb.fault.197
  FIMWB_198 : Subsystem  Tag=fimwb.fault.198
  FIMWB_199 : Subsystem  Tag=fimwb.fault.199
  FIMWB_200 : Subsystem  Tag=fimwb.fault.200
  FIMWB_201 : Subsystem  Tag=fimwb.fault.201
  FIMWB_202 : Subsystem  Tag=fimwb.fault.202
  FIMWB_203 : Subsystem  Tag=fimwb.fault.203
  FIMWB_204 : Subsystem  Tag=fimwb.fault.204
  FIMWB_205 : Subsystem  Tag=fimwb.fault.205
  FIMWB_309 : Subsystem  Tag=fimwb.fault.309
  FIMWB_310 : Subsystem  Tag=fimwb.fault.310
  FIMWB_311 : Subsystem  Tag=fimwb.fault.311
  FIMWB_312 : Subsystem  Tag=fimwb.fault.312
  FIMWB_351 : Subsystem  Tag=fimwb.fault.351
  FIMWB_352 : Subsystem  Tag=fimwb.fault.352
  FIMWB_353 : Subsystem  Tag=fimwb.fault.353
  MinMax : MinMax  Inputs=2  InputSameDT=on  SaturateOnIntegerOverflow=on
  Product : Product  Inputs=3  InputSameDT=on  RndMeth=Zero  SaturateOnIntegerOverflow=on  OutDataTypeStr=Inherit: Same as first input
  Product1 : Product  Inputs=*/  InputSameDT=on  RndMeth=Zero  SaturateOnIntegerOverflow=on  OutDataTypeStr=Inherit: Same as first input
  Product2 : Product  Inputs=/*  InputSameDT=on  RndMeth=Zero  SaturateOnIntegerOverflow=on  OutDataTypeStr=Inherit: Same as first input
  "Sonic Flow " : Constant  Value=1.0
  Sum : Sum  Inputs=+-|  InputSameDT=on  SaturateOnIntegerOverflow=on  OutDataTypeStr=Inherit: Same as first input
  Switch : Switch  Threshold=0.5
  f(theta) : Fcn  Expr=2.821 - 0.05231*u + 0.10299*u*u - 0.00063*u*u*u
  flow direction : Signum
  g(pratio) : Fcn  Expr=2*sqrt(u - u*u)
  "Throttle Flow, mdot (g/s)" : Outport  InitialOutput=0  VectorParamsAs1DForOutWhenUnconnected=off
  wires:
  Product/1 -> FIMWB_309/1(Original)
  Product1/1 -> FIMWB_310/1(Original)
  Product2/1 -> FIMWB_311/1(Original)
  Sum/1 -> FIMWB_312/1(Original)
  "Manifold Pressure, Pm (bar)"/1 -> FIMWB_351/1(Original)
  FIMWB_351/1(Result) -> FIMWB_189/1(Original), FIMWB_190/1(Original), FIMWB_191/1(Original)
  "Atmospheric Pressure, Pa (bar) "/1 -> FIMWB_352/1(Original)
  FIMWB_352/1(Result) -> FIMWB_192/1(Original), FIMWB_193/1(Original), FIMWB_194/1(Original)
  MinMax/1 -> FIMWB_353/1(Original)  "pratio"
  FIMWB_353/1(Result) -> FIMWB_195/1(Original), FIMWB_196/1(Original)
  "Throttle Angle, theta (deg)"/1 -> FIMWB_188/1(Original)
  FIMWB_188/1(Result) -> f(theta)/1
  FIMWB_189/1(Result) -> Product1/1, FIMWB_310/2(Operand1)
  FIMWB_190/1(Result) -> Product2/1, FIMWB_311/2(Operand1)
  FIMWB_191/1(Result) -> Sum/2, FIMWB_312/3(Operand2)
  FIMWB_192/1(Result) -> Product1/2, FIMWB_310/3(Operand2)
  FIMWB_193/1(Result) -> Product2/2, FIMWB_311/3(Operand2)
  FIMWB_194/1(Result) -> Sum/1, FIMWB_312/2(Operand1)
  FIMWB_195/1(Result) -> Switch/2
  FIMWB_196/1(Result) -> g(pratio)/1
  FIMWB_309/1(Result) -> FIMWB_197/1(Original)
  FIMWB_197/1(Result) -> "Throttle Flow, mdot (g/s)"/1
  FIMWB_310/1(Result) -> FIMWB_198/1(Original)
  FIMWB_198/1(Result) -> MinMax/1
  FIMWB_311/1(Result) -> FIMWB_199/1(Original)
  FIMWB_199/1(Result) -> MinMax/2
  "Sonic Flow "/1 -> FIMWB_200/1(Original)
  FIMWB_200/1(Result) -> Switch/3
  FIMWB_312/1(Result) -> FIMWB_201/1(Original)
  FIMWB_201/1(Result) -> flow direction/1
  Switch/1 -> FIMWB_202/1(Original)
  FIMWB_202/1(Result) -> Product/2, FIMWB_309/3(Operand2)
  f(theta)/1 -> FIMWB_203/1(Original)
  FIMWB_203/1(Result) -> Product/1, FIMWB_309/2(Operand1)
  flow direction/1 -> FIMWB_204/1(Original)
  FIMWB_204/1(Result) -> Product/3, FIMWB_309/4(Operand3)
  g(pratio)/1 -> FIMWB_205/1(Original)
  FIMWB_205/1(Result) -> Switch/1

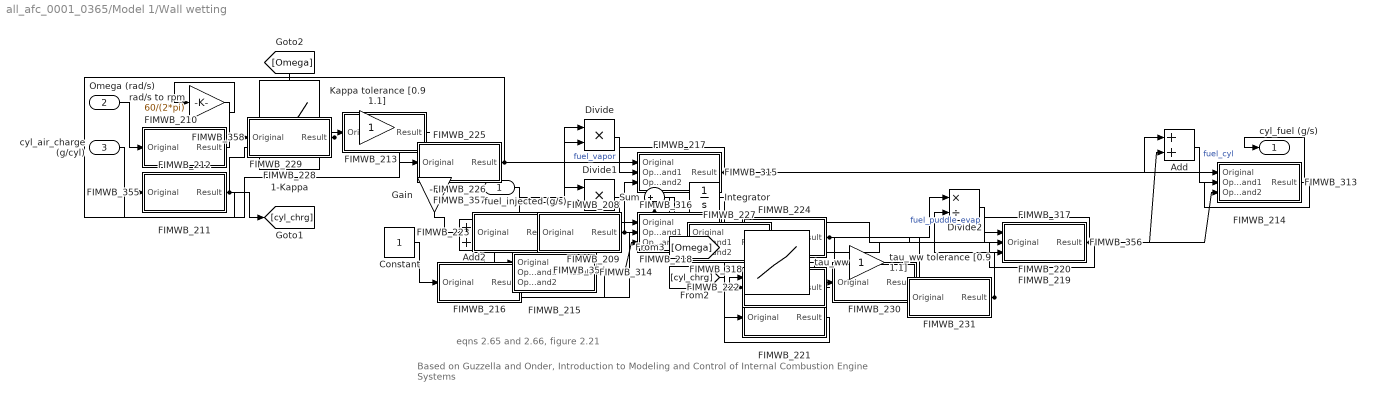
== system all_afc_0001_0365/Model 1/Wall wetting ==
  note: Based on Guzzella and Onder, Introduction to Modeling and Control of Internal Combustion Engine Systems
  note: eqns 2.65 and 2.66, figure 2.21
  fuel_injected (g/s) : Inport
  Omega (rad/s) : Inport  Port=2
  cyl_air_charge (g/cyl) : Inport  Port=3
  1-Kappa : Lookup_n-D  BreakpointsForDimension1=[1000,1500,2000,2500,3000]  BreakpointsForDimension2=[.1,.2,.3,.4]  Table=reshape([0.8,.7,.7,.8,.9,.7,.66,.65,.73,.85,.66,.66,.63,.66,.8,.6,.6,.6,.6,.7],5,4)  UseLastTableValue=on  RndMeth=Simplest
      settings: InputPortMap=u0,u1
  Add : Sum
  Add2 : Sum
  Constant : Constant
  Divide : Product  Inputs=**
  Divide1 : Product  Inputs=**
  Divide2 : Product  Inputs=*/
  FIMWB_208 : Subsystem  Tag=fimwb.fault.208
  FIMWB_209 : Subsystem  Tag=fimwb.fault.209
  FIMWB_210 : Subsystem  Tag=fimwb.fault.210
  FIMWB_211 : Subsystem  Tag=fimwb.fault.211
  FIMWB_212 : Subsystem  Tag=fimwb.fault.212
  FIMWB_213 : Subsystem  Tag=fimwb.fault.213
  FIMWB_214 : Subsystem  Tag=fimwb.fault.214
  FIMWB_215 : Subsystem  Tag=fimwb.fault.215
  FIMWB_216 : Subsystem  Tag=fimwb.fault.216
  FIMWB_217 : Subsystem  Tag=fimwb.fault.217
  FIMWB_218 : Subsystem  Tag=fimwb.fault.218
  FIMWB_219 : Subsystem  Tag=fimwb.fault.219
  FIMWB_220 : Subsystem  Tag=fimwb.fault.220
  FIMWB_221 : Subsystem  Tag=fimwb.fault.221
  FIMWB_222 : Subsystem  Tag=fimwb.fault.222
  FIMWB_223 : Subsystem  Tag=fimwb.fault.223
  FIMWB_224 : Subsystem  Tag=fimwb.fault.224
  FIMWB_225 : Subsystem  Tag=fimwb.fault.225
  FIMWB_226 : Subsystem  Tag=fimwb.fault.226
  FIMWB_227 : Subsystem  Tag=fimwb.fault.227
  FIMWB_228 : Subsystem  Tag=fimwb.fault.228
  FIMWB_229 : Subsystem  Tag=fimwb.fault.229
  FIMWB_230 : Subsystem  Tag=fimwb.fault.230
  FIMWB_231 : Subsystem  Tag=fimwb.fault.231
  FIMWB_313 : Subsystem  Tag=fimwb.fault.313
  FIMWB_314 : Subsystem  Tag=fimwb.fault.314
  FIMWB_315 : Subsystem  Tag=fimwb.fault.315
  FIMWB_316 : Subsystem  Tag=fimwb.fault.316
  FIMWB_317 : Subsystem  Tag=fimwb.fault.317
  FIMWB_318 : Subsystem  Tag=fimwb.fault.318
  FIMWB_354 : Subsystem  Tag=fimwb.fault.354
  FIMWB_355 : Subsystem  Tag=fimwb.fault.355
  FIMWB_356 : Subsystem  Tag=fimwb.fault.356
  FIMWB_357 : Subsystem  Tag=fimwb.fault.357
  FIMWB_358 : Subsystem  Tag=fimwb.fault.358
  Gain : Gain  Gain=-1
  Integrator : Integrator  InitialCondition=.0112
  Kappa tolerance [0.9 1.1] : Gain
  Sum : Sum  Inputs=|+-
  rad/s to rpm : Gain  Gain=60/(2*pi)
  tau_ww : Lookup_n-D  BreakpointsForDimension1=[1000,1500,2000,2500,3000]  BreakpointsForDimension2=[0.1,0.2,0.3,0.4]  Table=reshape([.4,.3,.35,.3,.2,.22,.22,.4,.35,.5,.20,.22,.5,.4,.35,.35,.3,.45,.5,.4],5,4)  UseLastTableValue=on  RndMeth=Simplest
      settings: InputPortMap=u0,u1
  tau_ww tolerance [0.9 1.1] : Gain
  cyl_fuel (g/s) : Outport  VectorParamsAs1DForOutWhenUnconnected=off
  wires:
  Add/1 -> FIMWB_313/1(Original)  "fuel_cyl"
  Add2/1 -> FIMWB_314/1(Original)
  Divide/1 -> FIMWB_315/1(Original)  "fuel_vapor"
  Divide1/1 -> FIMWB_316/1(Original)
  Divide2/1 -> FIMWB_317/1(Original)  "fuel_puddle_evap"
  Sum/1 -> FIMWB_318/1(Original)
  fuel_injected (g/s)/1 -> FIMWB_354/1(Original)
  FIMWB_354/1(Result) -> FIMWB_208/1(Original), FIMWB_209/1(Original)
  cyl_air_charge (g/cyl)/1 -> FIMWB_355/1(Original)
  FIMWB_355/1(Result) -> FIMWB_211/1(Original), FIMWB_212/1(Original)
  FIMWB_317/1(Result) -> FIMWB_356/1(Original)
  FIMWB_356/1(Result) -> FIMWB_219/1(Original), FIMWB_220/1(Original)
  Kappa tolerance [0.9 1.1]/1 -> FIMWB_357/1(Original)
  FIMWB_357/1(Result) -> FIMWB_225/1(Original), FIMWB_226/1(Original)
  rad/s to rpm/1 -> FIMWB_358/1(Original)
  FIMWB_358/1(Result) -> FIMWB_228/1(Original), FIMWB_229/1(Original)
  FIMWB_208/1(Result) -> Divide/2, FIMWB_315/3(Operand2)
  FIMWB_209/1(Result) -> Divide1/1, FIMWB_316/2(Operand1)
  Omega (rad/s)/1 -> FIMWB_210/1(Original)
  FIMWB_210/1(Result) -> rad/s to rpm/1
  FIMWB_211/1(Result) -> 1-Kappa/2
  FIMWB_212/1(Result) -> [cyl_chrg]
  1-Kappa/1 -> FIMWB_213/1(Original)
  FIMWB_213/1(Result) -> Kappa tolerance [0.9 1.1]/1
  FIMWB_313/1(Result) -> FIMWB_214/1(Original)
  FIMWB_214/1(Result) -> cyl_fuel (g/s)/1
  FIMWB_314/1(Result) -> FIMWB_215/1(Original)
  FIMWB_215/1(Result) -> Divide1/2, FIMWB_316/3(Operand2)
  Constant/1 -> FIMWB_216/1(Original)
  FIMWB_216/1(Result) -> Add2/2, FIMWB_314/3(Operand2)
  FIMWB_315/1(Result) -> FIMWB_217/1(Original)
  FIMWB_217/1(Result) -> Add/1, FIMWB_313/2(Operand1)
  FIMWB_316/1(Result) -> FIMWB_218/1(Original)
  FIMWB_218/1(Result) -> Sum/1, FIMWB_318/2(Operand1)
  FIMWB_219/1(Result) -> Add/2, FIMWB_313/3(Operand2)
  FIMWB_220/1(Result) -> Sum/2, FIMWB_318/3(Operand2)
  [cyl_chrg] -> FIMWB_221/1(Original)
  FIMWB_221/1(Result) -> tau_ww/2
  [Omega] -> FIMWB_222/1(Original)
  FIMWB_222/1(Result) -> tau_ww/1
  Gain/1 -> FIMWB_223/1(Original)
  FIMWB_223/1(Result) -> Add2/1, FIMWB_314/2(Operand1)
  Integrator/1 -> FIMWB_224/1(Original)
  FIMWB_224/1(Result) -> Divide2/1, FIMWB_317/2(Operand1)
  FIMWB_225/1(Result) -> Divide/1, FIMWB_315/2(Operand1)
  FIMWB_226/1(Result) -> Gain/1
  FIMWB_318/1(Result) -> FIMWB_227/1(Original)
  FIMWB_227/1(Result) -> Integrator/1
  FIMWB_228/1(Result) -> 1-Kappa/1
  FIMWB_229/1(Result) -> [Omega]
  tau_ww/1 -> FIMWB_230/1(Original)
  FIMWB_230/1(Result) -> tau_ww tolerance [0.9 1.1]/1
  tau_ww tolerance [0.9 1.1]/1 -> FIMWB_231/1(Original)
  FIMWB_231/1(Result) -> Divide2/2, FIMWB_317/3(Operand2)

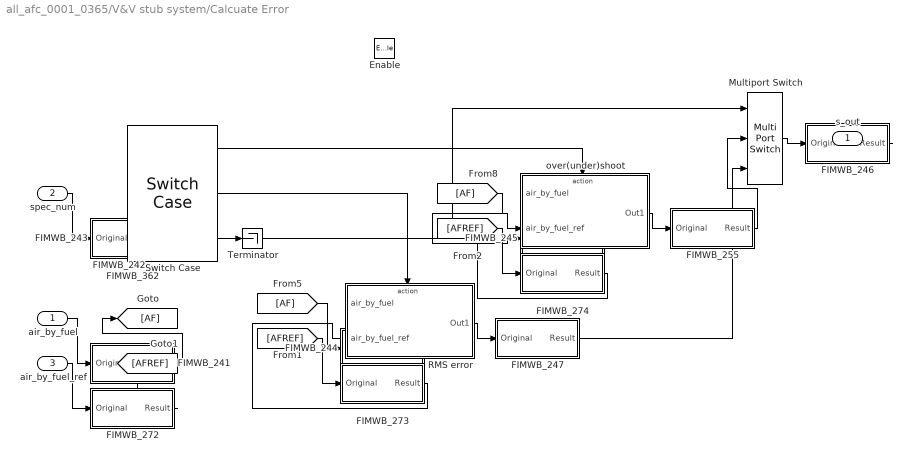
== system all_afc_0001_0365/V&V stub system/Calcuate Error ==
  "air_by_fuel " : Inport
  spec_num : Inport  Port=2  OutDataTypeStr=uint8
  air_by_fuel_ref : Inport  Port=3
  Enable : EnablePort
  FIMWB_241 : Subsystem  Tag=fimwb.fault.241
  FIMWB_242 : Subsystem  Tag=fimwb.fault.242
  FIMWB_243 : Subsystem  Tag=fimwb.fault.243
  FIMWB_244 : Subsystem  Tag=fimwb.fault.244
  FIMWB_245 : Subsystem  Tag=fimwb.fault.245
  FIMWB_246 : Subsystem  Tag=fimwb.fault.246
  FIMWB_247 : Subsystem  Tag=fimwb.fault.247
  FIMWB_255 : Subsystem  Tag=fimwb.fault.255
  FIMWB_272 : Subsystem  Tag=fimwb.fault.272
  FIMWB_273 : Subsystem  Tag=fimwb.fault.273
  FIMWB_274 : Subsystem  Tag=fimwb.fault.274
  FIMWB_362 : Subsystem  Tag=fimwb.fault.362
  Multiport Switch : MultiPortSwitch  Inputs=2  SaturateOnIntegerOverflow=off  InputSameDT=off
  RMS error : Subsystem  TreatAsAtomicUnit=on
  Switch Case : SwitchCase  CaseConditions={1,2}
  Terminator : Terminator
  over(under)shoot : Subsystem  TreatAsAtomicUnit=on
  "s_out " : Outport  VectorParamsAs1DForOutWhenUnconnected=off
  wires:
  Switch Case/1 -> over(under)shoot/Action
  Switch Case/2 -> RMS error/Action
  Switch Case/3 -> Terminator/1
  spec_num/1 -> FIMWB_362/1(Original)
  FIMWB_362/1(Result) -> FIMWB_242/1(Original), FIMWB_243/1(Original)
  "air_by_fuel "/1 -> FIMWB_241/1(Original)
  FIMWB_241/1(Result) -> [AF]
  FIMWB_242/1(Result) -> Multiport Switch/1
  FIMWB_243/1(Result) -> Switch Case/1
  [AF] -> FIMWB_244/1(Original)
  FIMWB_244/1(Result) -> RMS error/1("air_by_fuel ")
  [AF] -> FIMWB_245/1(Original)
  FIMWB_245/1(Result) -> over(under)shoot/1("air_by_fuel ")
  Multiport Switch/1 -> FIMWB_246/1(Original)
  FIMWB_246/1(Result) -> "s_out "/1
  RMS error/1(Out1) -> FIMWB_247/1(Original)
  FIMWB_247/1(Result) -> Multiport Switch/3
  over(under)shoot/1(Out1) -> FIMWB_255/1(Original)
  FIMWB_255/1(Result) -> Multiport Switch/2
  air_by_fuel_ref/1 -> FIMWB_272/1(Original)
  FIMWB_272/1(Result) -> [AFREF]
  [AFREF] -> FIMWB_273/1(Original)
  FIMWB_273/1(Result) -> RMS error/2(air_by_fuel_ref)
  [AFREF] -> FIMWB_274/1(Original)
  FIMWB_274/1(Result) -> over(under)shoot/2(air_by_fuel_ref)

== system all_afc_0001_0365/V&V stub system/FIMWB_239 ==
  Original : Inport
  Result : Outport
  wires:
  Original/1 -> Result/1

== system all_afc_0001_0365/V&V stub system/FIMWB_240 ==
  Original : Inport
  Result : Outport
  wires:
  Original/1 -> Result/1

== system all_afc_0001_0365/V&V stub system/FIMWB_260 ==
  Original : Inport
  Result : Outport
  wires:
  Original/1 -> Result/1

== system all_afc_0001_0365/V&V stub system/FIMWB_261 ==
  Original : Inport
  Result : Outport
  wires:
  Original/1 -> Result/1

== system all_afc_0001_0365/V&V stub system/FIMWB_265 ==
  Original : Inport
  Result : Outport
  wires:
  Original/1 -> Result/1

== system all_afc_0001_0365/V&V stub system/FIMWB_275 ==
  Original : Inport
  Result : Outport
  wires:
  Original/1 -> Result/1

== system all_afc_0001_0365/V&V stub system/FIMWB_276 ==
  Original : Inport
  Result : Outport
  wires:
  Original/1 -> Result/1

== system all_afc_0001_0365/Model 1/AF_Controller/FIMWB_014 ==
  Original : Inport
  Result : Outport
  wires:
  Original/1 -> Result/1

== system all_afc_0001_0365/Model 1/AF_Controller/FIMWB_015 ==
  Original : Inport
  Result : Outport
  wires:
  Original/1 -> Result/1

== system all_afc_0001_0365/Model 1/AF_Controller/FIMWB_016 ==
  Original : Inport
  Result : Outport
  wires:
  Original/1 -> Result/1

== system all_afc_0001_0365/Model 1/AF_Controller/FIMWB_017 ==
  Original : Inport
  Result : Outport
  wires:
  Original/1 -> Result/1

== system all_afc_0001_0365/Model 1/AF_Controller/FIMWB_018 ==
  Original : Inport
  Result : Outport
  wires:
  Original/1 -> Result/1

== system all_afc_0001_0365/Model 1/AF_Controller/FIMWB_019 ==
  Original : Inport
  Result : Outport
  wires:
  Original/1 -> Result/1

== system all_afc_0001_0365/Model 1/AF_Controller/FIMWB_020 ==
  Original : Inport
  Result : Outport
  wires:
  Original/1 -> Result/1

== system all_afc_0001_0365/Model 1/AF_Controller/FIMWB_262 ==
  Original : Inport
  Result : Outport
  wires:
  Original/1 -> Result/1

== system all_afc_0001_0365/Model 1/AF_Controller/FIMWB_269 ==
  Original : Inport
  Result : Outport
  wires:
  Original/1 -> Result/1

== system all_afc_0001_0365/Model 1/AF_Controller/fuel_controller ==
  note: Global Inputs
  note: Trigger Layer
  trigger_pwon : Inport
  trigger_10ms : Inport  Port=2
  engine_speed : Inport  Port=3
  throttle_angle_deg : Inport  Port=4
  throttle_flow : Inport  Port=5
  airbyfuel_meas : Inport  Port=6
  DataStoreMemory : DataStoreMemory  DataStoreName=engine_speed  ShowAdditionalParam=off  OutDataTypeStr=single
      settings: AttributesFormatString=engine speed
  DataStoreMemory1 : DataStoreMemory  DataStoreName=throttle_flow  ShowAdditionalParam=off  OutDataTypeStr=single
      settings: AttributesFormatString=throttle flow
  DataStoreMemory2 : DataStoreMemory  DataStoreName=airbyfuel_meas  ShowAdditionalParam=off  OutDataTypeStr=single
      settings: AttributesFormatString=lambda_meas
  DataStoreMemory3 : DataStoreMemory  DataStoreName=throttle_angle  ShowAdditionalParam=off  OutDataTypeStr=single
      settings: AttributesFormatString=throttle flow
  DataStoreWrite : DataStoreWrite  Priority=1  DataStoreName=engine_speed  IndexOptions=Index vector (dialog)  Indices=1  OutputSizes=1
  DataStoreWrite1 : DataStoreWrite  Priority=1  DataStoreName=throttle_flow  IndexOptions=Index vector (dialog)  Indices=1  OutputSizes=1
  DataStoreWrite2 : DataStoreWrite  Priority=1  DataStoreName=airbyfuel_meas  IndexOptions=Index vector (dialog)  Indices=1  OutputSizes=1
  DataStoreWrite3 : DataStoreWrite  Priority=1  DataStoreName=throttle_angle  IndexOptions=Index vector (dialog)  Indices=1  OutputSizes=1
  FIMWB_021 : Subsystem  Tag=fimwb.fault.21
  FIMWB_022 : Subsystem  Tag=fimwb.fault.22
  FIMWB_023 : Subsystem  Tag=fimwb.fault.23
  FIMWB_024 : Subsystem  Tag=fimwb.fault.24
  fuel_controller_10ms : Subsystem  Priority=30  TreatAsAtomicUnit=on
      settings: AttributesFormatString=Priority = %<Priority>
  fuel_controller_mode_10ms : Subsystem  Priority=20  TreatAsAtomicUnit=on
      settings: AttributesFormatString=Priority = %<Priority>
  fuel_controller_pwon : Subsystem  Priority=10  TreatAsAtomicUnit=on
      settings: AttributesFormatString=Priority = %<Priority>
  wires:
  trigger_10ms/1 -> fuel_controller_mode_10ms/Trigger, fuel_controller_10ms/Trigger
  trigger_pwon/1 -> fuel_controller_pwon/Trigger
  engine_speed/1 -> FIMWB_021/1(Original)
  FIMWB_021/1(Result) -> DataStoreWrite/1
  throttle_angle_deg/1 -> FIMWB_022/1(Original)
  FIMWB_022/1(Result) -> DataStoreWrite3/1
  throttle_flow/1 -> FIMWB_023/1(Original)
  FIMWB_023/1(Result) -> DataStoreWrite1/1
  airbyfuel_meas/1 -> FIMWB_024/1(Original)
  FIMWB_024/1(Result) -> DataStoreWrite2/1
